simulink model "Mission_Server_QDrone_YOLO_Landing_Diagnostics"  (R2021b)
settings: Solver=ode2  StartTime=0.0  StopTime=inf  FixedStep=0.001  RelTol=1e-3  EnableMultiTasking=on
undefined symbols (not defined in the file): Host, qc_get_step_size
libraries: quarc_library x21, simulink x4
settings Model: SimulationMode=external  ExtModeTrigDuration=10000  Creator=Admin  LastModifiedBy=user
settings SolverCC: AlgebraicLoopSolver=TrustRegion  PositivePriorityOrder=on
settings DataIOCC: ReturnWorkspaceOutputs=off
settings DebuggingCC: SFUnexpectedBacktrackingDiag=warning  SFNoUnconditionalDefaultTransitionDiag=warning  SFExecutionAtInitializationDiag=none  SFMachineParentedDataDiag=warning  ArithmeticOperatorsInVariantConditions=warning
settings SFSimCC: SimUseLocalCustomCode=off  CustomCodeUndefinedFunction=UseInterfaceOnly
settings RTWCC: Description=QUARC Win64 Target Using Toolchain  SystemTargetFile=quarc_win64.tlc  TemplateMakefile=quarc_default_tmf  RTWUseLocalCustomCode=off  Toolchain=QUARC win64 | nmake (64-bit Windows)  BuildConfiguration=Faster Runs
settings CodeAppCC: StateflowObjectComments=on
settings STFCustomTargetCC: ConcurrentExecutionCompliant=on  UseToolchainInfoCompliant=on  SystemTargetFile=quarc_win64.tlc
settings GRTTargetCC: TargetLangStandard=C89/C90 (ANSI)  ParMdlRefBuildCompliant=off  CompOptLevelCompliant=off  CombineOutputUpdateFcns=off  MatFileLogging=off  CPPClassGenCompliant=off  GRTInterface=on  ExtMode=on  ExtModeMexFile=quarc_comm  ExtModeMexArgs='-w -d %d -uri %u -URI_Follower tcpip://localhost:18001'
settings ConfigComp: CovMetricSettings=dw  CovSaveCumulativeToWorkspaceVar=on  CovSaveSingleToWorkspaceVar=on  CovExternalEMLEnable=off

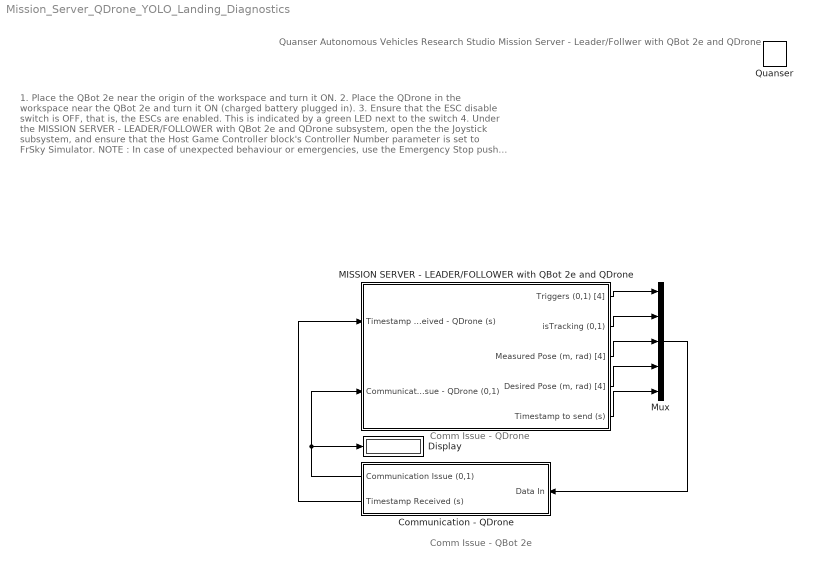
== system Mission_Server_QDrone_YOLO_Landing_Diagnostics ==
  note: 1. Place the QBot 2e near the origin of the workspace and turn it ON.
      | 2. Place the QDrone in the workspace near the QBot 2e and turn it ON (charged battery plugged in).
      | 3. Ensure that the ESC disable switch is OFF, that is, the ESCs are enabled. This is indicated by a green LED next to the switch
      | 4. Under the MISSION SERVER - LEADER/FOLLOWER with QBot 2e and QDrone subsystem, open the the Joystick subsystem, and ensure that the Host Game Controller block's Controller Number parameter is set to FrSky Simulator.
      | NOTE : In case of unexpected behaviour or emergencies, use the Emergency Stop push button on the Spektrum Joystick to cut all power to the motors (this will result in the drone falling).
      | 5. Open the Data Server (Localization) subsystem and follow the steps there to set up the correct calibration and rigid body definition files for the selected QBot 2e and QDrone.
      | 6. Under the QUARC menu, click on Build .
      | 7. Under the QUARC menu, click on Start . Wait for the model to start running (takes ~1 to 5 seconds for the Motive API to initialize and send localization data).
      | 8. In the MISSION SERVER - LEADER/FOLLOWER with QBot 2e and QDrone subsystem, ensure that the isTracking? display shows 1 and that the Joystick Issue display shows 0 (joystick must be powered ON with USB dongle attached to the PC).
      | 9. Start running the Joystick_Stabilizer_QBot2e_Leader.mdl model.
      | 10. Start running the Commander_Stabilizer_QDrone_Follower.mdl model.
      | 11. Arm the drone by moving the Arm/Disarm toggle to the 2 position.
      | 12. Takeoff the drone by moving the Takeoff/Land toggle to the 2 position. The QDrone should takeoff and hover.
      | 13. Drive the QBot 2e around using the joystick handset. Use the RIGHT stick (Roll/Pitch) to drive the QBot 2e forward/backward and turning/yawing.
      | 14. When finished, move the Takeoff/Land toggle to the 0 position to land the drone. The QDrone should land.
      | 15. Move the Arm/Disarm toggle to the 0 position. (the Commander_Stabilizer_QDrone_Follower.mdl model disarms the drone and stops automatically upon landing).
      | 16. Stop the QBot 2e model. Then stop this model.
  note: Quanser Autonomous Vehicles Research Studio
      | Mission Server - Leader/Follwer with QBot 2e and QDrone
  note: Comm Issue - QDrone
  note: Comm Issue - QBot 2e
  Communication - QDrone : Subsystem
  Display : Display
  MISSION SERVER - LEADER/FOLLOWER with QBot 2e and QDrone : Subsystem
  Mux : Mux  Inputs=5
  Quanser : quarc_library/Logos/Quanser
  wires:
  Communication - QDrone/2(Timestamp Received (s)) -> MISSION SERVER - LEADER/FOLLOWER with QBot 2e and QDrone/1(Timestamp Received - QDrone (s))
  MISSION SERVER - LEADER/FOLLOWER with QBot 2e and QDrone/5(Timestamp to send (s)) -> Mux/5
  Mux/1 -> Communication - QDrone/1(Data In)
  Communication - QDrone/1(Communication Issue (0,1)) -> Display/1, MISSION SERVER - LEADER/FOLLOWER with QBot 2e and QDrone/2(Communication Issue - QDrone (0,1))
  MISSION SERVER - LEADER/FOLLOWER with QBot 2e and QDrone/3("Measured Pose (m, rad) [4]") -> Mux/3
  MISSION SERVER - LEADER/FOLLOWER with QBot 2e and QDrone/4("Desired Pose (m, rad) [4]") -> Mux/4
  MISSION SERVER - LEADER/FOLLOWER with QBot 2e and QDrone/1(Triggers (0,1) [4]) -> Mux/1
  MISSION SERVER - LEADER/FOLLOWER with QBot 2e and QDrone/2(isTracking (0,1)) -> Mux/2

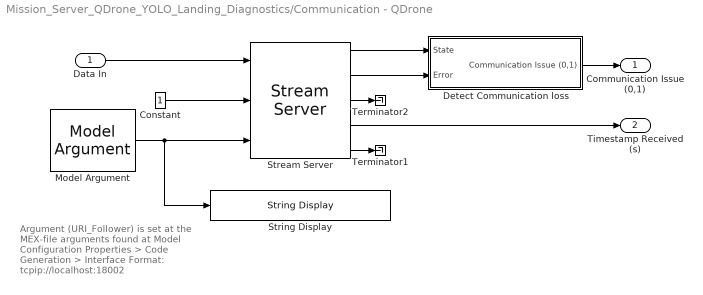
== system Mission_Server_QDrone_YOLO_Landing_Diagnostics/Communication - QDrone ==
  note: Argument (URI_Follower) is set at the MEX-file arguments found at Model Configuration Properties > Code Generation > Interface
      |
      | Format:
      | tcpip://localhost:18002
  Data In : Inport
  Constant : Constant
  Detect Communication loss : Subsystem
  Model Argument : quarc_library/Sources/Signals/Model Argument  argument_name=URI_Follower  has_value=on  data_type_mode=Specify via dialog  data_type=char  max_length=80  default_value=0  variable_size=off
      settings: AttributesFormatString=(-%<argument_name>)  SourceProductName=QUARC Targets
  Stream Server : quarc_library/Communications/Basic/Stream Server  uri_source=External input port  uri=tcpip://localhost:18877  send_buffer_size=1460  receive_buffer_size=1460  byte_order=little endian (Intel - LSB first)  optimization=Minimum latency  send_options=Send most recent data  receive_options=Receive most recent data  default_value=zeros(1,1)  sample_time=qc_get_step_size  active=off  implementation=Use blocking I/O in a separate thread  send_fifo_size=1000  receive_fifo_size=1000  send_priority=0  receive_priority=0  send_dimensions=off  receive_dimensions=off  max_dimensions=-1  data_type=Inherited via back propagation  type_expr=BusObject
  "String Display " : quarc_library/Strings/String Display  alignment=center  display_mode=Single line  sample_time=-1  use_new=off
      settings: SourceProductName=QUARC Targets
  Terminator1 : Terminator
  Terminator2 : Terminator
  Communication Issue (0,1) : Outport  VectorParamsAs1DForOutWhenUnconnected=off
  Timestamp Received (s) : Outport  Port=2  VectorParamsAs1DForOutWhenUnconnected=off
  wires:
  Constant/1 -> Stream Server/2
  Data In/1 -> Stream Server/1
  Stream Server/3 -> Terminator2/1
  Stream Server/5 -> Terminator1/1
  Model Argument/1 -> "String Display "/1, Stream Server/3
  Stream Server/4 -> Timestamp Received (s)/1
  Stream Server/1 -> Detect Communication loss/1(State)
  Stream Server/2 -> Detect Communication loss/2(Error)
  Detect Communication loss/1(Communication Issue (0,1)) -> Communication Issue (0,1)/1

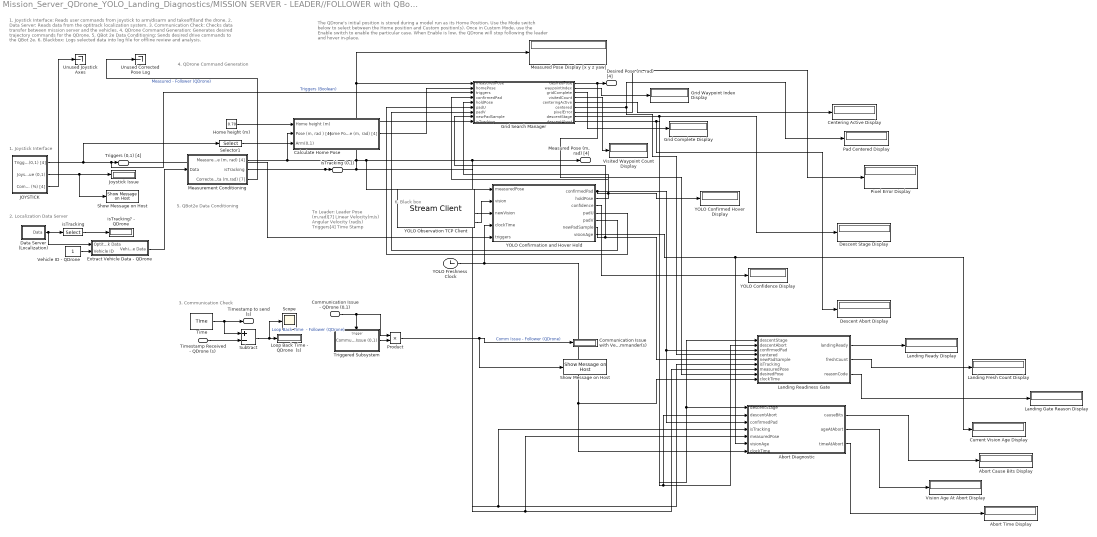
== system Mission_Server_QDrone_YOLO_Landing_Diagnostics/MISSION SERVER - LEADER//FOLLOWER with QBot 2e and QDrone ==
  note: To Leader:
      | Leader Pose (m,rad)[7]
      | Linear Velocity(m/s)
      | Angular Velocity (rad/s)
      | Triggers[4]
      | Time Stamp
  note: 5. QBot2e Data Conditioning
  note: The QDrone's initial position is stored during a model run as its Home Position.
      | Use the Mode switch below to select between the Home position and Custom position(s).
      | Once in Custom Mode, use the Enable switch to enable the particular case.
      | When Enable is low, the QDrone will stop following the leader and hover in-place.
  note: 3. Communication Check
  note: 6. Black box
  note: 2. Localization Data Server
  note: 1. Joystick Interface
  note: 4. QDrone Command Generation
  note: 1. Joystick Interface: Reads user commands from joystick to arm/disarm and takeoff/land the drone.
      | 2. Data Server: Reads data from the optitrack localization system.
      | 3. Communication Check: Checks data transfer between mission server and the vehicles.
      | 4. QDrone Command Generation: Generates desired trajectory commands for the QDrone.
      | 5. QBot 2e Data Conditioning: Sends desired drive commands to the QBot 2e.
      | 6. Blackbox: Logs selected data into log file for offline review and analysis.
  Timestamp Received - QDrone (s) : Inport
  Communication Issue - QDrone (0,1) : Inport  Port=2
  Abort Cause Bits Display : Display
  Abort Diagnostic : MATLAB Function  TreatAsAtomicUnit=on
  Abort Time Display : Display
  Calculate Home Pose : Subsystem
  Centering Active Display : Display
  Communication Issue with Vehicle Commander(s) : Display
  Current Vision Age Display : Display
  "Data Server (Localization) " : Subsystem
  Descent Abort Display : Display
  Descent Stage Display : Display
  Extract Vehicle Data - QDrone : Subsystem
  Grid Complete Display : Display
  Grid Search Manager : MATLAB Function  TreatAsAtomicUnit=on
  Grid Waypoint Index Display : Display
  Home height (m) : Constant  Value=0.70
  JOYSTICK : Subsystem
  Joystick Issue : Display
  Landing Fresh Count Display : Display
  Landing Gate Reason Display : Display
  Landing Readiness Gate : MATLAB Function  TreatAsAtomicUnit=on
  Landing Ready Display : Display
  Loop Back Time - QDrone  (s) : Display
  Measured Pose Display [x y z yaw] : Display
  Measurement Conditioning : Subsystem
  Pad Centered Display : Display
  Pixel Error Display : Display
  Product : Product
  Scope : Scope
  Selector1 : Selector  InputPortWidth=4  IndexOptions=Index vector (dialog)  Indices=[1]  OutputSizes=1
  Show Message on Host : quarc_library/Sinks/Error Handling/Show Message on Host  message_type=Fixed error message  message_icon=Warning  message=Mission Server: Communication Issue with remote vehicle(s)
      settings: AttributesFormatString="\"%<message>\""  SourceProductName=QUARC Targets
  "Show Message on Host " : quarc_library/Sinks/Error Handling/Show Message on Host  message_type=Fixed error message  message_icon=Warning  message=Mission Server: Joystick Disconnected
      settings: AttributesFormatString="\"%<message>\""  SourceProductName=QUARC Targets
  Subtract : Sum  Inputs=+-
  Time : quarc_library/Sources/Time/Time  time_source=Wall clock  sample_time=qc_get_step_size
  Triggered Subsystem : Subsystem  TreatAsAtomicUnit=on
  Unused Corrected Pose Log : Terminator
  Unused Joystick Axes : Terminator
  Vehicle ID - QDrone : Constant
  Vision Age At Abort Display : Display
  Visited Waypoint Count Display : Display
  YOLO Confidence Display : Display
  YOLO Confirmation and Hover Hold : MATLAB Function  TreatAsAtomicUnit=on
  YOLO Confirmed Hover Display : Display
  YOLO Freshness Clock : Clock
  YOLO Observation TCP Client : quarc_library/Communications/Basic/Stream Client  uri_source=Specify via dialog (do not evaluate)  uri=tcpip://localhost:18901  send_buffer_size=1460  receive_buffer_size=1460  byte_order=little endian (Intel - LSB first)  optimization=Minimum latency  send_options=Do not send data  receive_options=Receive most recent data  default_value=[0 0 0 0 -1 0]  sample_time=qc_get_step_size  active=off  implementation=Use blocking I/O in a separate thread  send_fifo_size=1000  receive_fifo_size=1000  send_priority=0  receive_priority=0  send_dimensions=off  receive_dimensions=off  max_dimensions=-1  data_type=Inherited via back propagation  type_expr=BusObject
      settings: AttributesFormatString="\"tcpip://localhost:18901\""
  isTracking : Selector  InputPortWidth=7  IndexOptions=Index vector (dialog)  Indices=[7]  OutputSizes=1
  isTracking? - QDrone : Display
  Triggers (0,1) [4] : Outport  VectorParamsAs1DForOutWhenUnconnected=off
  isTracking (0,1) : Outport  Port=2  VectorParamsAs1DForOutWhenUnconnected=off
  "Measured Pose (m, rad) [4]" : Outport  Port=3  VectorParamsAs1DForOutWhenUnconnected=off
  "Desired Pose (m, rad) [4]" : Outport  Port=4  VectorParamsAs1DForOutWhenUnconnected=off
  Timestamp to send (s) : Outport  Port=5  VectorParamsAs1DForOutWhenUnconnected=off
  wires:
  Communication Issue - QDrone (0,1)/1 -> Product/1, Triggered Subsystem/Trigger
  isTracking/1 -> isTracking? - QDrone/1
  JOYSTICK/2(Joystick Issue (0,1)) -> Joystick Issue/1, "Show Message on Host "/1
  Time/1 -> Timestamp to send (s)/1, Subtract/1
  Timestamp Received - QDrone (s)/1 -> Subtract/2
  Subtract/1 -> Loop Back Time - QDrone  (s)/1, Scope/1  "Loop Back Time  - Follower (QDrone)"
  Measurement Conditioning/2(isTracking) -> Landing Readiness Gate/6(isTracking), Abort Diagnostic/4(isTracking), Grid Search Manager/9(isTracking), isTracking (0,1)/1
  Measurement Conditioning/1("Measured Pose (m, rad) [4]") -> Landing Readiness Gate/7(measuredPose), Abort Diagnostic/5(measuredPose), "Measured Pose (m, rad) [4]"/1, YOLO Confirmation and Hover Hold/1(measuredPose), Measured Pose Display [x y z yaw]/1, Grid Search Manager/1(measuredPose), Calculate Home Pose/2("Pose (m, rad ) [4]")
  "Data Server (Localization) "/1(Data) -> isTracking/1, Extract Vehicle Data - QDrone/1(Optitrack Data)
  Vehicle ID - QDrone/1 -> Extract Vehicle Data - QDrone/2(Vehicle ID)
  Calculate Home Pose/1("Home Pose (m, rad) [4]") -> Grid Search Manager/2(homePose)
  Home height (m)/1 -> Calculate Home Pose/1(Home height (m))
  Triggered Subsystem/1(Communication Issue (0,1)) -> Product/2
  Product/1 -> Communication Issue with Vehicle Commander(s)/1, Show Message on Host/1  "Comm Issue - Follower (QDrone)"
  Extract Vehicle Data - QDrone/1(Vehicle Data) -> Measurement Conditioning/1(Data)
  JOYSTICK/1(Triggers (0,1) [4]) -> YOLO Confirmation and Hover Hold/5(triggers), Grid Search Manager/3(triggers), Triggers (0,1) [4]/1, Selector1/1  "Triggers (Boolean)"
  JOYSTICK/3(Commands (%) [4]) -> Unused Joystick Axes/1
  Selector1/1 -> Calculate Home Pose/3(Arm(0,1))
  Measurement Conditioning/3(Corrected Pose Data (m,rad) [7]) -> Unused Corrected Pose Log/1  "Measured - Follower (QDrone)"
  Grid Search Manager/1(desiredPose) -> "Desired Pose (m, rad) [4]"/1, Landing Readiness Gate/8(desiredPose)
  Grid Search Manager/2(waypointIndex) -> Grid Waypoint Index Display/1
  Grid Search Manager/3(gridComplete) -> Grid Complete Display/1
  Grid Search Manager/4(visitedCount) -> Visited Waypoint Count Display/1
  YOLO Observation TCP Client/3 -> YOLO Confirmation and Hover Hold/2(vision)
  YOLO Observation TCP Client/4 -> YOLO Confirmation and Hover Hold/3(newVision)
  YOLO Freshness Clock/1 -> Abort Diagnostic/7(clockTime), Landing Readiness Gate/9(clockTime), YOLO Confirmation and Hover Hold/4(clockTime)
  YOLO Confirmation and Hover Hold/1(confirmedPad) -> Landing Readiness Gate/3(confirmedPad), Abort Diagnostic/3(confirmedPad), Grid Search Manager/4(confirmedPad), YOLO Confirmed Hover Display/1
  YOLO Confirmation and Hover Hold/2(holdPose) -> Grid Search Manager/5(holdPose)
  YOLO Confirmation and Hover Hold/3(confidence) -> YOLO Confidence Display/1
  YOLO Confirmation and Hover Hold/4(padU) -> Grid Search Manager/6(padU)
  YOLO Confirmation and Hover Hold/5(padV) -> Grid Search Manager/7(padV)
  YOLO Confirmation and Hover Hold/6(newPadSample) -> Grid Search Manager/8(newPadSample), Landing Readiness Gate/5(newPadSample)
  Grid Search Manager/5(centeringActive) -> Centering Active Display/1
  Grid Search Manager/6(centered) -> Pad Centered Display/1, Landing Readiness Gate/4(centered)
  Grid Search Manager/7(pixelError) -> Pixel Error Display/1
  Grid Search Manager/8(descentStage) -> Landing Readiness Gate/1(descentStage), Abort Diagnostic/1(descentStage), Descent Stage Display/1
  Grid Search Manager/9(descentAbort) -> Abort Diagnostic/2(descentAbort), Landing Readiness Gate/2(descentAbort), Descent Abort Display/1
  Landing Readiness Gate/1(landingReady) -> Landing Ready Display/1
  Landing Readiness Gate/2(freshCount) -> Landing Fresh Count Display/1
  Landing Readiness Gate/3(reasonCode) -> Landing Gate Reason Display/1
  YOLO Confirmation and Hover Hold/7(visionAge) -> Abort Diagnostic/6(visionAge), Current Vision Age Display/1
  Abort Diagnostic/1(causeBits) -> Abort Cause Bits Display/1
  Abort Diagnostic/2(ageAtAbort) -> Vision Age At Abort Display/1
  Abort Diagnostic/3(timeAtAbort) -> Abort Time Display/1

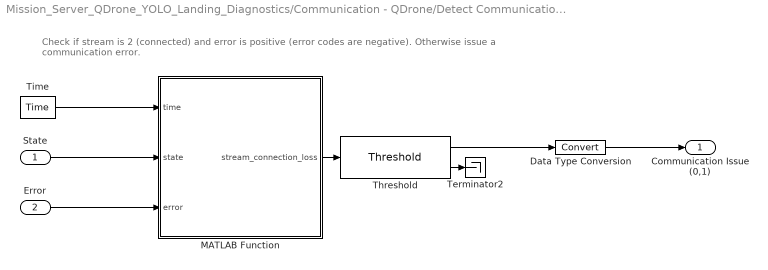
== system Mission_Server_QDrone_YOLO_Landing_Diagnostics/Communication - QDrone/Detect Communication loss ==
  note: Check if stream is 2 (connected) and error is positive (error codes are negative). Otherwise issue a communication error.
  State : Inport
  Error : Inport  Port=2
  Data Type Conversion : DataTypeConversion
  MATLAB Function : MATLAB Function  TreatAsAtomicUnit=on
  Terminator2 : Terminator
  Threshold : quarc_library/Discontinuities/Threshold  operator=>=  param_src=Specify via dialog  threshold=0.5  duration=0.1
      settings: SourceProductName=QUARC Targets
  Time : quarc_library/Sources/Time/Time  time_source=Wall clock  sample_time=qc_get_step_size
  Communication Issue (0,1) : Outport  VectorParamsAs1DForOutWhenUnconnected=off
  wires:
  Error/1 -> MATLAB Function/3(error)
  MATLAB Function/1(stream_connection_loss) -> Threshold/1
  State/1 -> MATLAB Function/2(state)
  Time/1 -> MATLAB Function/1(time)
  Threshold/2 -> Terminator2/1
  Data Type Conversion/1 -> Communication Issue (0,1)/1
  Threshold/1 -> Data Type Conversion/1

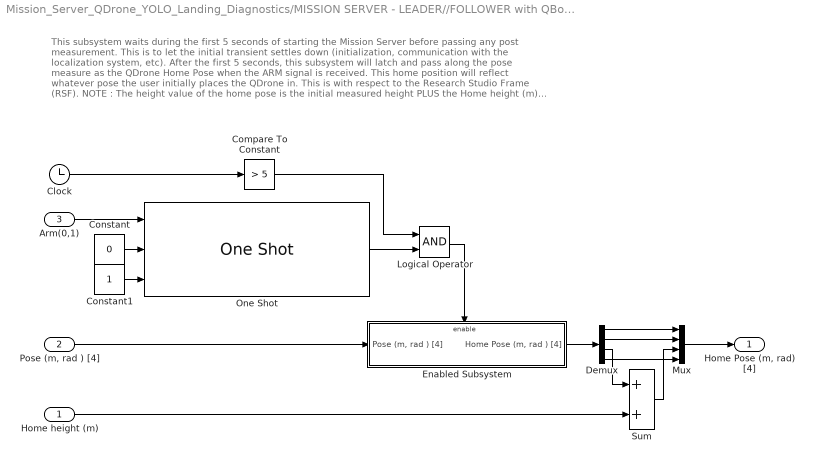
== system Mission_Server_QDrone_YOLO_Landing_Diagnostics/MISSION SERVER - LEADER//FOLLOWER with QBot 2e and QDrone/Calculate Home Pose ==
  note: This subsystem waits during the first 5 seconds of starting the Mission Server before passing any post measurement.
      | This is to let the initial transient settles down (initialization, communication with the localization system, etc).
      | After the first 5 seconds, this subsystem will latch and pass along the pose measure as the QDrone Home Pose when
      | the ARM signal is received.
      | This home position will reflect whatever pose the user initially places the QDrone in.
      | This is with respect to the Research Studio Frame (RSF).
      |
      | NOTE : The height value of the home pose is the initial measured height PLUS the Home height (m) input value.
  Home height (m) : Inport
  "Pose (m, rad ) [4]" : Inport  Port=2
  Arm(0,1) : Inport  Port=3
  Clock : Clock
  Compare To Constant : simulink/Logic and Bit Operations/Compare To Constant  relop=>  const=5  OutDataTypeStr=boolean
  Constant : Constant  Value=0
  Constant1 : Constant
  Demux : Demux
  Enabled Subsystem : Subsystem  TreatAsAtomicUnit=on
  Logical Operator : Logic  AllPortsSameDT=off  OutDataTypeStr=boolean
  Mux : Mux
  One Shot : quarc_library/Discontinuities/One Shot  trigger_type=Rising edge  redun_pulse=Ignore extraneous pulse  width_source=Specify via dialog  pulse_width=1/qc_get_step_size
      settings: SourceProductName=QUARC Targets
  Sum : Sum
  "Home Pose (m, rad) [4]" : Outport  VectorParamsAs1DForOutWhenUnconnected=off
  wires:
  Constant/1 -> One Shot/2
  Constant1/1 -> One Shot/3
  Arm(0,1)/1 -> One Shot/1
  One Shot/1 -> Logical Operator/2
  "Pose (m, rad ) [4]"/1 -> Enabled Subsystem/1("Pose (m, rad ) [4] ")
  Clock/1 -> Compare To Constant/1
  Compare To Constant/1 -> Logical Operator/1
  Logical Operator/1 -> Enabled Subsystem/Enable
  Enabled Subsystem/1("Home Pose (m, rad ) [4]") -> Demux/1
  Demux/1 -> Mux/1
  Demux/2 -> Mux/2
  Demux/4 -> Mux/4
  Demux/3 -> Sum/1
  Sum/1 -> Mux/3
  Home height (m)/1 -> Sum/2
  Mux/1 -> "Home Pose (m, rad) [4]"/1

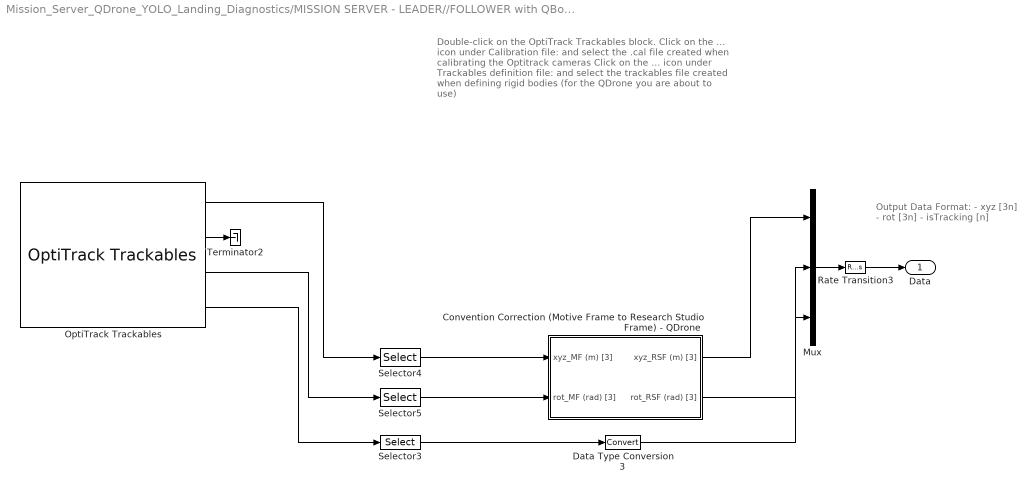
== system Mission_Server_QDrone_YOLO_Landing_Diagnostics/MISSION SERVER - LEADER//FOLLOWER with QBot 2e and QDrone/Data Server (Localization)  ==
  note: Output Data Format:
      | - xyz [3n]
      | - rot [3n]
      | - isTracking [n]
  note: Double-click on the OptiTrack Trackables block.
      |
      | Click on the ... icon under Calibration file: and select the .cal file
      | created when calibrating the Optitrack cameras
      |
      | Click on the ... icon under Trackables definition file: and select
      | the trackables file created when defining rigid bodies (for the
      | QDrone you are about to use)
  Convention Correction (Motive Frame to Research Studio Frame) - QDrone : Subsystem
  Data Type Conversion3 : DataTypeConversion
  Mux : Mux  Inputs=3
  OptiTrack Trackables : quarc_library/Devices/Third-Party/NaturalPoint/OptiTrack/OptiTrack Trackables  calibration_file=C:\Users\user\Documents\OptiTrack\Session 2026-09-15\Calibration Exceptional (MeanErr 0.544 mm) 2026-09-15 10.cal  rigid_body_file=C:\Users\user\Documents\OptiTrack\Session 2026-09-15\RigidBody 01.tra  rigid_body_ids=1  sample_time=qc_get_step_size*10  active=off
      settings: SourceProductName=QUARC Targets
  Rate Transition3 : RateTransition
  Selector3 : Selector  InputPortWidth=1  IndexOptions=Index vector (dialog)  Indices=[1]  OutputSizes=1
  Selector4 : Selector  InputPortWidth=3  IndexOptions=Index vector (dialog)  Indices=[1:3]  OutputSizes=1
  Selector5 : Selector  InputPortWidth=3  IndexOptions=Index vector (dialog)  Indices=[1:3]  OutputSizes=1
  Terminator2 : Terminator
  Data : Outport  VectorParamsAs1DForOutWhenUnconnected=off
  wires:
  OptiTrack Trackables/2 -> Terminator2/1
  OptiTrack Trackables/4 -> Selector3/1
  OptiTrack Trackables/3 -> Selector5/1
  Selector3/1 -> Data Type Conversion3/1
  OptiTrack Trackables/1 -> Selector4/1
  Selector4/1 -> Convention Correction (Motive Frame to Research Studio Frame) - QDrone/1(xyz_MF (m) [3])
  Selector5/1 -> Convention Correction (Motive Frame to Research Studio Frame) - QDrone/2(rot_MF (rad) [3])
  Mux/1 -> Rate Transition3/1
  Rate Transition3/1 -> Data/1
  Convention Correction (Motive Frame to Research Studio Frame) - QDrone/1(xyz_RSF (m) [3]) -> Mux/1
  Convention Correction (Motive Frame to Research Studio Frame) - QDrone/2(rot_RSF (rad) [3]) -> Mux/2
  Data Type Conversion3/1 -> Mux/3

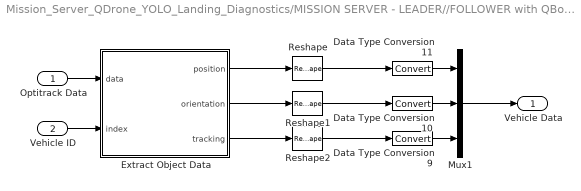
== system Mission_Server_QDrone_YOLO_Landing_Diagnostics/MISSION SERVER - LEADER//FOLLOWER with QBot 2e and QDrone/Extract Vehicle Data - QDrone ==
  Optitrack Data : Inport
  Vehicle ID : Inport  Port=2
  Data Type Conversion10 : DataTypeConversion
  Data Type Conversion11 : DataTypeConversion
  Data Type Conversion9 : DataTypeConversion
  Extract Object Data : MATLAB Function  TreatAsAtomicUnit=on
  Mux1 : Mux  Inputs=3
  Reshape : Reshape
  Reshape1 : Reshape
  Reshape2 : Reshape
  Vehicle Data : Outport  VectorParamsAs1DForOutWhenUnconnected=off
  wires:
  Reshape2/1 -> Data Type Conversion9/1
  Reshape1/1 -> Data Type Conversion10/1
  Reshape/1 -> Data Type Conversion11/1
  Data Type Conversion9/1 -> Mux1/3
  Data Type Conversion10/1 -> Mux1/2
  Data Type Conversion11/1 -> Mux1/1
  Extract Object Data/2(orientation) -> Reshape1/1
  Extract Object Data/3(tracking) -> Reshape2/1
  Extract Object Data/1(position) -> Reshape/1
  Mux1/1 -> Vehicle Data/1
  Optitrack Data/1 -> Extract Object Data/1(data)
  Vehicle ID/1 -> Extract Object Data/2(index)

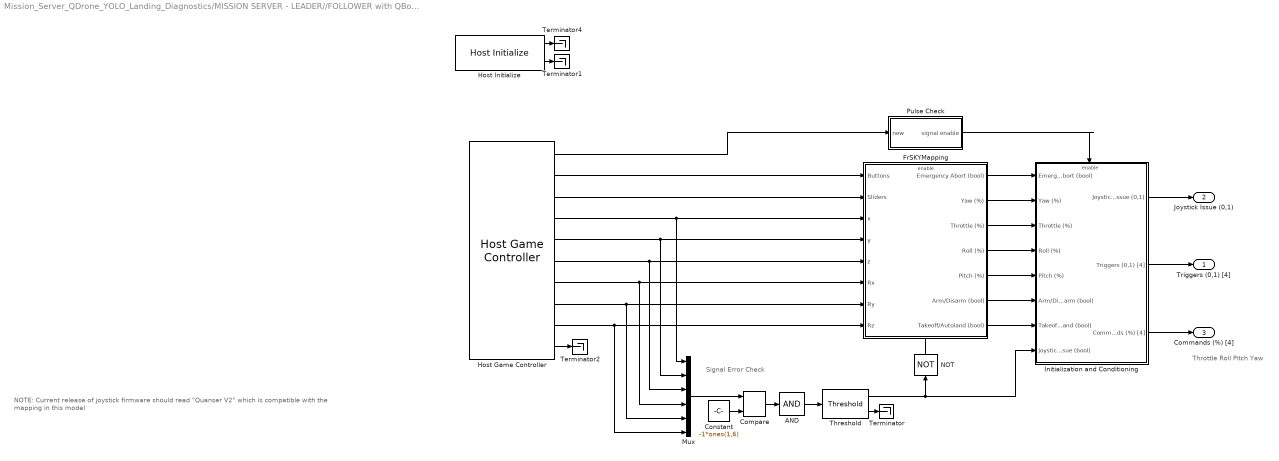
== system Mission_Server_QDrone_YOLO_Landing_Diagnostics/MISSION SERVER - LEADER//FOLLOWER with QBot 2e and QDrone/JOYSTICK ==
  note: Throttle
      | Roll
      | Pitch
      | Yaw
  note: Signal Error Check
  note: NOTE: Current release of joystick firmware should read "Quanser V2" which is compatible with the mapping in this model
  AND : Logic  Inputs=1  AllPortsSameDT=off  OutDataTypeStr=boolean
  Compare : quarc_library/Logic Operations/Compare  operator===  output_data_type=boolean
      settings: SourceProductName=QUARC Targets
  Constant : Constant  Value=-1*ones(1,6)
  FrSKYMapping : Subsystem
  Host Game Controller : quarc_library/Devices/Peripherals/Host/Host Game Controller  object_name=Host-1  controller=1  buffer_size=20  deadzone=[]  saturation=[]  sample_time=qc_get_step_size  auto_center=off  enabled=on  debug_mode=off
      settings: SourceProductName=QUARC Targets
  Host Initialize : quarc_library/Devices/Peripherals/Host/Host Initialize  object_name=Host-1  uri_source=Use external mode communications  uri=tcpip://localhost:18001  send_buffer_size=1000  receive_buffer_size=1000  thread_priority=0  run_client=on  use_window=off  window_position=[]  sample_time=qc_get_step_size  active=on
      settings: SourceProductName=QUARC Targets
  Initialization and Conditioning : Subsystem  TreatAsAtomicUnit=on
  Mux : Mux  Inputs=6
  NOT : Logic  Operator=NOT  IconShape=distinctive  AllPortsSameDT=off  OutDataTypeStr=boolean
  Pulse Check : Subsystem  TreatAsAtomicUnit=on
  Terminator{,1..2,4} (4 alike) : Terminator
  Threshold : quarc_library/Discontinuities/Threshold  operator=>=  param_src=Specify via dialog  threshold=0.5  duration=0.2
      settings: SourceProductName=QUARC Targets
  Triggers (0,1) [4] : Outport  VectorParamsAs1DForOutWhenUnconnected=off
  Joystick Issue (0,1) : Outport  Port=2  VectorParamsAs1DForOutWhenUnconnected=off
  Commands (%) [4] : Outport  Port=3  VectorParamsAs1DForOutWhenUnconnected=off
  wires:
  Initialization and Conditioning/1(Joystick Issue (0,1)) -> Joystick Issue (0,1)/1
  Host Game Controller/10 -> Terminator2/1
  Host Initialize/1 -> Terminator4/1
  Host Initialize/2 -> Terminator1/1
  Initialization and Conditioning/2(Triggers (0,1) [4]) -> Triggers (0,1) [4]/1
  Initialization and Conditioning/3(Commands (%) [4]) -> Commands (%) [4]/1
  AND/1 -> Threshold/1
  NOT/1 -> FrSKYMapping/Enable
  Threshold/1 -> Initialization and Conditioning/8(Joystick Issue (bool)), NOT/1
  Host Game Controller/3 -> FrSKYMapping/2(Sliders)
  Host Game Controller/2 -> FrSKYMapping/1(Buttons)
  Threshold/2 -> Terminator/1
  Compare/1 -> AND/1
  Constant/1 -> Compare/2
  Mux/1 -> Compare/1
  Host Game Controller/9 -> FrSKYMapping/8(Rz), Mux/6
  Host Game Controller/8 -> FrSKYMapping/7(Ry), Mux/5
  Host Game Controller/7 -> FrSKYMapping/6(Rx), Mux/4
  Host Game Controller/6 -> FrSKYMapping/5(z), Mux/3
  Host Game Controller/5 -> FrSKYMapping/4(y), Mux/2
  Host Game Controller/4 -> FrSKYMapping/3(x), Mux/1
  FrSKYMapping/7(Takeoff/Autoland (bool)) -> Initialization and Conditioning/7(Takeoff/AutoLand (bool))
  Pulse Check/1(signal enable) -> Initialization and Conditioning/Enable
  Host Game Controller/1 -> Pulse Check/1(new)
  FrSKYMapping/4(Roll (%)) -> Initialization and Conditioning/4(Roll (%))
  FrSKYMapping/6("Arm/Disarm (bool) ") -> Initialization and Conditioning/6(Arm/Disarm (bool))
  FrSKYMapping/5(Pitch (%)) -> Initialization and Conditioning/5(Pitch (%))
  FrSKYMapping/1(Emergency Abort (bool)) -> Initialization and Conditioning/1(Emergency Abort (bool))
  FrSKYMapping/3(Throttle (%)) -> Initialization and Conditioning/3(Throttle (%))
  FrSKYMapping/2(Yaw (%)) -> Initialization and Conditioning/2(Yaw (%))

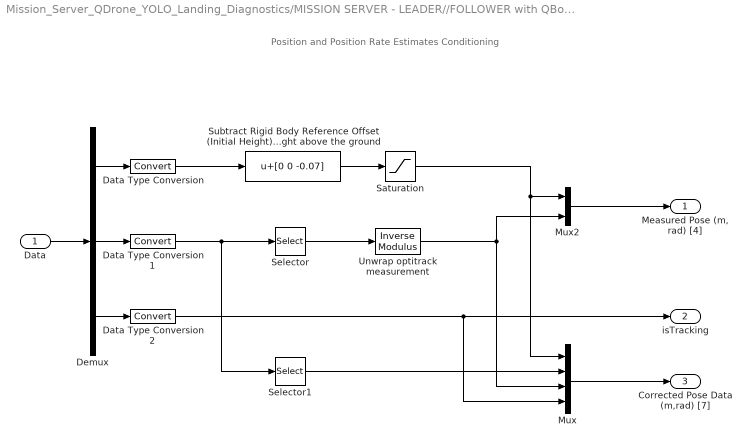
== system Mission_Server_QDrone_YOLO_Landing_Diagnostics/MISSION SERVER - LEADER//FOLLOWER with QBot 2e and QDrone/Measurement Conditioning ==
  note: Position and Position Rate Estimates Conditioning
  Data : Inport
  Data Type Conversion : DataTypeConversion
  Data Type Conversion1 : DataTypeConversion
  Data Type Conversion2 : DataTypeConversion
  Demux : Demux  Outputs=[3 3 1]
  Mux : Mux
  Mux2 : Mux  Inputs=[3 1]
  Saturation : Saturate  UpperLimit=[2 2 5]  LowerLimit=[-2 -2 0]
  Selector : Selector  InputPortWidth=3  IndexOptions=Index vector (dialog)  Indices=[3]  OutputSizes=1
  Selector1 : Selector  InputPortWidth=3  IndexOptions=Index vector (dialog)  Indices=[1 2]  OutputSizes=1
  Subtract Rigid Body Reference Offset (Initial Height) to get height above the ground : Bias  Bias=[0 0 -0.07]
  Unwrap optitrack measurement : quarc_library/Discontinuities/Inverse Modulus  modulus=2*pi  output_derivative=off  output_revolutions=off  max_x=Inf  min_x=-Inf
  "Measured Pose (m, rad) [4]" : Outport  VectorParamsAs1DForOutWhenUnconnected=off
  isTracking : Outport  Port=2  VectorParamsAs1DForOutWhenUnconnected=off
  Corrected Pose Data (m,rad) [7] : Outport  Port=3  VectorParamsAs1DForOutWhenUnconnected=off
  wires:
  Demux/2 -> Data Type Conversion1/1
  Demux/1 -> Data Type Conversion/1
  Demux/3 -> Data Type Conversion2/1
  Mux2/1 -> "Measured Pose (m, rad) [4]"/1
  Data/1 -> Demux/1
  Data Type Conversion2/1 -> Mux/4, isTracking/1
  Subtract Rigid Body Reference Offset (Initial Height) to get height above the ground/1 -> Saturation/1
  Saturation/1 -> Mux2/1, Mux/1
  Data Type Conversion1/1 -> Selector1/1, Selector/1
  Selector/1 -> Unwrap optitrack measurement/1
  Data Type Conversion/1 -> Subtract Rigid Body Reference Offset (Initial Height) to get height above the ground/1
  Unwrap optitrack measurement/1 -> Mux/3, Mux2/2
  Mux/1 -> Corrected Pose Data (m,rad) [7]/1
  Selector1/1 -> Mux/2

== system Mission_Server_QDrone_YOLO_Landing_Diagnostics/MISSION SERVER - LEADER//FOLLOWER with QBot 2e and QDrone/Triggered Subsystem ==
  note: This looks for the first falling edge of the communication issue before allowing a communication issue to be triggered,
      | because the mission server model starts first.
  Trigger : TriggerPort  TriggerType=falling  VariantControl=Variant
  Add : Sum
  Compare To Constant : simulink/Logic and Bit Operations/Compare To Constant  relop=>=  const=1  OutDataTypeStr=boolean
  Constant : Constant
  Memory : Memory  InheritSampleTime=on
  Communication Issue (0,1) : Outport  InitialOutput=0  VectorParamsAs1DForOutWhenUnconnected=off
  wires:
  Constant/1 -> Add/1
  Memory/1 -> Add/2
  Add/1 -> Compare To Constant/1, Memory/1
  Compare To Constant/1 -> Communication Issue (0,1)/1

== system Mission_Server_QDrone_YOLO_Landing_Diagnostics/MISSION SERVER - LEADER//FOLLOWER with QBot 2e and QDrone/Calculate Home Pose/Enabled Subsystem ==
  "Pose (m, rad ) [4] " : Inport
  Enable : EnablePort
  "Home Pose (m, rad ) [4]" : Outport  VectorParamsAs1DForOutWhenUnconnected=off
  wires:
  "Pose (m, rad ) [4] "/1 -> "Home Pose (m, rad ) [4]"/1

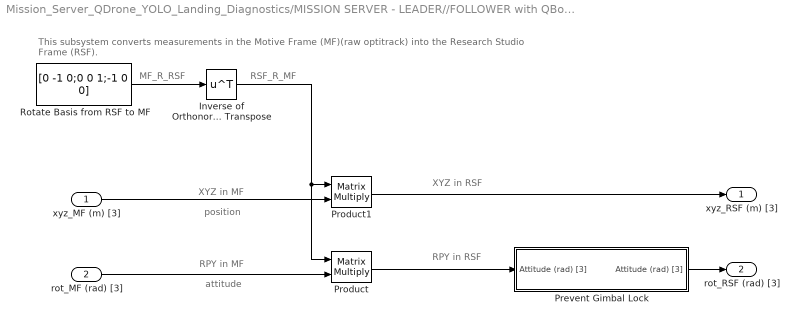
== system Mission_Server_QDrone_YOLO_Landing_Diagnostics/MISSION SERVER - LEADER//FOLLOWER with QBot 2e and QDrone/Data Server (Localization) /Convention Correction (Motive Frame to Research Studio Frame) - QDrone ==
  note: MF_R_RSF
  note: This subsystem converts measurements in the Motive Frame (MF)(raw optitrack) into the Research Studio Frame (RSF).
  note: RSF_R_MF
  note: XYZ in MF
  note: RPY in MF
  note: position
  note: attitude
  note: XYZ in RSF
  note: RPY in RSF
  xyz_MF (m) [3] : Inport
  rot_MF (rad) [3] : Inport  Port=2
  Inverse of Orthonormal Matrix is its Transpose : Math  Operator=transpose  SignedPower=on  SaturateOnIntegerOverflow=on
  Prevent Gimbal Lock : Subsystem
  Product : Product  Multiplication=Matrix(*)
  Product1 : Product  Multiplication=Matrix(*)
  Rotate Basis from RSF to MF : Constant  Value=[0 -1 0;0 0 1;-1 0 0]
  xyz_RSF (m) [3] : Outport  VectorParamsAs1DForOutWhenUnconnected=off
  rot_RSF (rad) [3] : Outport  Port=2  VectorParamsAs1DForOutWhenUnconnected=off
  wires:
  Rotate Basis from RSF to MF/1 -> Inverse of Orthonormal Matrix is its Transpose/1
  xyz_MF (m) [3]/1 -> Product1/2
  Inverse of Orthonormal Matrix is its Transpose/1 -> Product1/1, Product/1
  rot_MF (rad) [3]/1 -> Product/2
  Product1/1 -> xyz_RSF (m) [3]/1
  Product/1 -> Prevent Gimbal Lock/1(Attitude (rad) [3])
  Prevent Gimbal Lock/1("Attitude (rad) [3] ") -> rot_RSF (rad) [3]/1

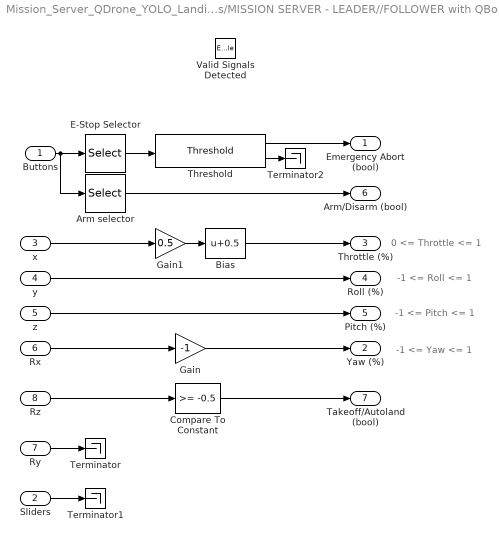
== system Mission_Server_QDrone_YOLO_Landing_Diagnostics/MISSION SERVER - LEADER//FOLLOWER with QBot 2e and QDrone/JOYSTICK/FrSKYMapping ==
  note: -1 <= Pitch <= 1
  note: -1 <= Roll <= 1
  note: 0 <= Throttle <= 1
  note: -1 <= Yaw <= 1
  Buttons : Inport
  Sliders : Inport  Port=2
  x : Inport  Port=3
  y : Inport  Port=4
  z : Inport  Port=5
  Rx : Inport  Port=6
  Ry : Inport  Port=7
  Rz : Inport  Port=8
  Valid Signals Detected : EnablePort
  Arm selector : Selector  InputPortWidth=32  IndexOptions=Index vector (dialog)  Indices=[2]  OutputSizes=1
  Bias : Bias  Bias=0.5
  Compare To Constant : simulink/Logic and Bit Operations/Compare To Constant  relop=>=  const=-0.5  OutDataTypeStr=boolean
  E-Stop Selector : Selector  InputPortWidth=32  IndexOptions=Index vector (dialog)  Indices=[1]  OutputSizes=1
  Gain : Gain  Gain=-1
  Gain1 : Gain  Gain=0.5
  Terminator : Terminator
  Terminator1 : Terminator
  Terminator2 : Terminator
  Threshold : quarc_library/Discontinuities/Threshold  operator=>=  param_src=Specify via dialog  threshold=0.5  duration=0.2
      settings: SourceProductName=QUARC Targets
  Emergency Abort (bool) : Outport  VectorParamsAs1DForOutWhenUnconnected=off
  Yaw (%) : Outport  Port=2  VectorParamsAs1DForOutWhenUnconnected=off
  Throttle (%) : Outport  Port=3  VectorParamsAs1DForOutWhenUnconnected=off
  Roll (%) : Outport  Port=4  VectorParamsAs1DForOutWhenUnconnected=off
  Pitch (%) : Outport  Port=5  VectorParamsAs1DForOutWhenUnconnected=off
  "Arm/Disarm (bool) " : Outport  Port=6  VectorParamsAs1DForOutWhenUnconnected=off
  Takeoff/Autoland (bool) : Outport  Port=7  VectorParamsAs1DForOutWhenUnconnected=off
  wires:
  Bias/1 -> Throttle (%)/1
  Gain1/1 -> Bias/1
  Gain/1 -> Yaw (%)/1
  Threshold/2 -> Terminator2/1
  Threshold/1 -> Emergency Abort (bool)/1
  Compare To Constant/1 -> Takeoff/Autoland (bool)/1
  Rz/1 -> Compare To Constant/1
  E-Stop Selector/1 -> Threshold/1
  Sliders/1 -> Terminator1/1
  Ry/1 -> Terminator/1
  Rx/1 -> Gain/1
  z/1 -> Pitch (%)/1
  y/1 -> Roll (%)/1
  x/1 -> Gain1/1
  Arm selector/1 -> "Arm/Disarm (bool) "/1
  Buttons/1 -> E-Stop Selector/1, Arm selector/1

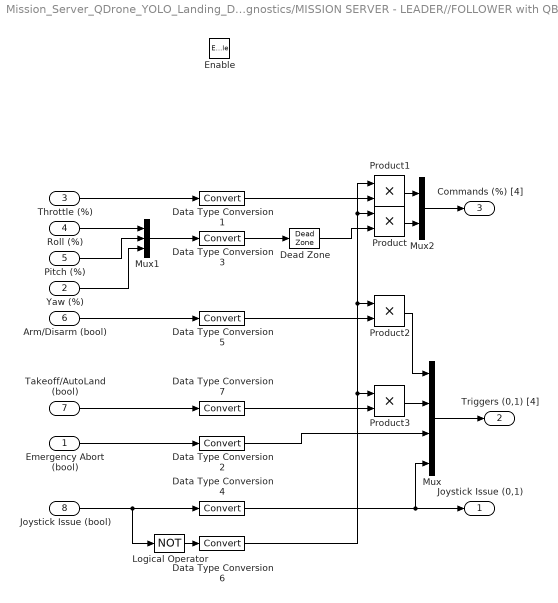
== system Mission_Server_QDrone_YOLO_Landing_Diagnostics/MISSION SERVER - LEADER//FOLLOWER with QBot 2e and QDrone/JOYSTICK/Initialization and Conditioning ==
  Emergency Abort (bool) : Inport
  Yaw (%) : Inport  Port=2
  Throttle (%) : Inport  Port=3
  Roll (%) : Inport  Port=4
  Pitch (%) : Inport  Port=5
  Arm/Disarm (bool) : Inport  Port=6
  Takeoff/AutoLand (bool) : Inport  Port=7
  Joystick Issue (bool) : Inport  Port=8
  Enable : EnablePort  StatesWhenEnabling=reset
  Data Type Conversion{1..7} (7 alike) : DataTypeConversion
  Dead Zone : DeadZone  LowerValue=-0.01  UpperValue=0.01  SaturateOnIntegerOverflow=on
  Logical Operator : Logic  Operator=NOT  AllPortsSameDT=off  OutDataTypeStr=boolean
  Mux : Mux
  Mux1 : Mux  Inputs=3
  Mux2 : Mux  Inputs=2
  Product{,1..3} (4 alike) : Product
  Joystick Issue (0,1) : Outport  InitialOutput=0  VectorParamsAs1DForOutWhenUnconnected=off
  Triggers (0,1) [4] : Outport  Port=2  InitialOutput=0  VectorParamsAs1DForOutWhenUnconnected=off
  Commands (%) [4] : Outport  Port=3  InitialOutput=0  VectorParamsAs1DForOutWhenUnconnected=off
  wires:
  Mux2/1 -> Commands (%) [4]/1
  Data Type Conversion7/1 -> Product3/2
  Product3/1 -> Mux/2
  Takeoff/AutoLand (bool)/1 -> Data Type Conversion7/1
  Data Type Conversion5/1 -> Product2/2
  Product2/1 -> Mux/1
  Data Type Conversion6/1 -> Product3/1, Product2/1, Product/1, Product1/1
  Dead Zone/1 -> Product/2
  Data Type Conversion1/1 -> Product1/2
  Product1/1 -> Mux2/1
  Product/1 -> Mux2/2
  Logical Operator/1 -> Data Type Conversion6/1
  Data Type Conversion2/1 -> Mux/3
  Mux/1 -> Triggers (0,1) [4]/1
  Arm/Disarm (bool)/1 -> Data Type Conversion5/1
  Data Type Conversion3/1 -> Dead Zone/1
  Emergency Abort (bool)/1 -> Data Type Conversion2/1
  Data Type Conversion4/1 -> Joystick Issue (0,1)/1, Mux/4
  Yaw (%)/1 -> Mux1/3
  Pitch (%)/1 -> Mux1/2
  Roll (%)/1 -> Mux1/1
  Throttle (%)/1 -> Data Type Conversion1/1
  Mux1/1 -> Data Type Conversion3/1
  Joystick Issue (bool)/1 -> Logical Operator/1, Data Type Conversion4/1

== system Mission_Server_QDrone_YOLO_Landing_Diagnostics/MISSION SERVER - LEADER//FOLLOWER with QBot 2e and QDrone/JOYSTICK/Pulse Check ==
  note: For this subsystem we will count the number of new pulses. The data can be considered enabled once the count of new signals has gone beyond 1. This will enable the Initializing and conditioning subsystem.
  new : Inport
  Compare : quarc_library/Logic Operations/Compare  operator=>=  output_data_type=boolean
      settings: SourceProductName=QUARC Targets
  Pulse Check : Constant
  "pulse count " : Subsystem  TreatAsAtomicUnit=on
  signal enable : Outport  InitialOutput=0  VectorParamsAs1DForOutWhenUnconnected=off
  wires:
  Compare/1 -> signal enable/1
  Pulse Check/1 -> Compare/2
  new/1 -> "pulse count "/Trigger
  "pulse count "/1(Number of Pulses) -> Compare/1

== system Mission_Server_QDrone_YOLO_Landing_Diagnostics/MISSION SERVER - LEADER//FOLLOWER with QBot 2e and QDrone/Data Server (Localization) /Convention Correction (Motive Frame to Research Studio Frame) - QDrone/Prevent Gimbal Lock ==
  note: Remapping the rotation order to prevent gimbal lock
      | in heading/yaw due to Euler singularity condition
  Attitude (rad) [3] : Inport
  Demux : Demux  Outputs=3
  Euler Angles from Rotation Matrix (Relative ZYX) : quarc_library/Math Operations/Matrices/Euler Angles from Rotation Matrix  menu_order=Relative Z-Y-X
      settings: SourceProductName=QUARC Targets
  Euler Angles to Rotation Matrix (Relative YZX) : quarc_library/Math Operations/Matrices/Euler Angles to Rotation Matrix  menu_order=Relative Y-Z-X
      settings: SourceProductName=QUARC Targets
  Mux : Mux  Inputs=3
  "Attitude (rad) [3] " : Outport  VectorParamsAs1DForOutWhenUnconnected=off
  wires:
  Euler Angles from Rotation Matrix (Relative ZYX)/2 -> Mux/2
  Euler Angles from Rotation Matrix (Relative ZYX)/1 -> Mux/3
  Euler Angles from Rotation Matrix (Relative ZYX)/3 -> Mux/1
  Euler Angles to Rotation Matrix (Relative YZX)/1 -> Euler Angles from Rotation Matrix (Relative ZYX)/1
  Attitude (rad) [3]/1 -> Demux/1
  Mux/1 -> "Attitude (rad) [3] "/1
  Demux/2 -> Euler Angles to Rotation Matrix (Relative YZX)/1
  Demux/3 -> Euler Angles to Rotation Matrix (Relative YZX)/2
  Demux/1 -> Euler Angles to Rotation Matrix (Relative YZX)/3

== system Mission_Server_QDrone_YOLO_Landing_Diagnostics/MISSION SERVER - LEADER//FOLLOWER with QBot 2e and QDrone/JOYSTICK/Pulse Check/pulse count  ==
  Trigger : TriggerPort  TriggerType=either  VariantControl=Variant
  Constant1 : Constant  Value=0
  Increment Stored Integer : simulink/Additional Math & Discrete/Additional Math: Increment - Decrement/Increment Stored Integer
  Sum : Sum  Inputs=|++
  Unit Delay : UnitDelay  SampleTime=-1  HasFrameUpgradeWarning=on
  Number of Pulses : Outport  VectorParamsAs1DForOutWhenUnconnected=off
  wires:
  Constant1/1 -> Sum/1
  Sum/1 -> Increment Stored Integer/1
  Unit Delay/1 -> Sum/2
  Increment Stored Integer/1 -> Unit Delay/1, Number of Pulses/1

== matlab function Mission_Server_QDrone_YOLO_Landing_Diagnostics/MISSION SERVER - LEADER//FOLLOWER with QBot 2e and QDrone/Grid Search Manager ==
  data: measuredPose input; desiredPose output; homePose input; triggers input; waypointIndex output; gridComplete output; visitedCount output; confirmedPad input; holdPose input; padU input; padV input; newPadSample input; centeringActive output; centered output; pixelError output; isTracking input; descentStage output; descentAbort output
function [desiredPose,waypointIndex,gridComplete,visitedCount,centeringActive,centered,pixelError,descentStage,descentAbort] = fcn(measuredPose,homePose,triggers,confirmedPad,holdPose,padU,padV,newPadSample,isTracking)
%#codegen
% Stage 0: search; 1: center at 0.70; 2: descend to 0.60;
% 3: center at 0.60; 4: descend to 0.55; 5: low hover.
persistent stage dwell takeoffWasLow reverseOrder complete visited sessionActive centerMode centerPose centerOrigin centerGood descentMode abortLatched
if isempty(stage)
 stage=uint8(0);dwell=uint16(0);takeoffWasLow=true;reverseOrder=false;
 complete=false;visited=uint8(0);sessionActive=false;centerMode=false;
 centerPose=zeros(4,1);centerOrigin=zeros(2,1);centerGood=uint8(0);
 descentMode=uint8(0);abortLatched=false;
end
takeoff=triggers(2)>0.5;
wps=[-1.2 -1 0.7;-0.6 -1 0.7;0 -1 0.7;0.6 -1 0.7;1.2 -1 0.7;1.2 -0.333333 0.7;0.6 -0.333333 0.7;0 -0.333333 0.7;-0.6 -0.333333 0.7;-1.2 -0.333333 0.7;-1.2 0.333333 0.7;-0.6 0.333333 0.7;0 0.333333 0.7;0.6 0.333333 0.7;1.2 0.333333 0.7;1.2 1 0.7;0.6 1 0.7;0 1 0.7;-0.6 1 0.7;-1.2 1 0.7];
baseMap=[0.00163 0.00019;7e-05 -0.00166];
cameraOffset=[0.11;0];
imageCenter=[320;240];
pixelError=zeros(2,1);
validPose=all(isfinite(measuredPose)) && all(isfinite(homePose));
if ~takeoff
 stage=uint8(0);dwell=uint16(0);takeoffWasLow=true;reverseOrder=false;
 sessionActive=false;centerMode=false;centerGood=uint8(0);
 descentMode=uint8(0);abortLatched=false;
elseif ~sessionActive
 complete=false;visited=uint8(0);sessionActive=true;
end
if takeoff && confirmedPad && isTracking>0.5 && validPose && ~centerMode
 centerMode=true;centerPose=holdPose;centerPose(3)=0.70;
 centerOrigin=holdPose(1:2);centerGood=uint8(0);descentMode=uint8(1);
end
desiredPose=homePose;desiredPose(3)=0.70;
if centerMode
 if isTracking<=0.5 || ~validPose || ~confirmedPad || measuredPose(3)<0.45
  abortLatched=true;centerGood=uint8(0);
  if validPose && isTracking>0.5
   centerPose(3)=min(max(measuredPose(3),0.55),0.70);
  end
 end
 if ~abortLatched
  h=min(max(measuredPose(3),0.50),0.70);
  map=baseMap*(h/0.70);
  target=imageCenter-map\cameraOffset;
  pixelError=[padU-target(1);padV-target(2)];
  if newPadSample
   if norm(pixelError)<=20
    if centerGood<uint8(10),centerGood=centerGood+uint8(1);end
   else
    centerGood=uint8(0);
    bodyStep=map*pixelError;
    a=measuredPose(4)-0.015;
    R=[cos(a) -sin(a);sin(a) cos(a)];
    step=R*bodyStep;n=norm(step);
    if n>0.005,step=step*(0.005/n);end
    candidate=centerPose(1:2)+step;
    offset=candidate-centerOrigin;on=norm(offset);
    if on>0.5,candidate=centerOrigin+offset*(0.5/on);end
    xLim=[-1.2 1.2];yLim=[-1 1];
    centerPose(1)=min(max(candidate(1),xLim(1)),xLim(2));
    centerPose(2)=min(max(candidate(2),yLim(1)),yLim(2));
   end
   xyError=norm(measuredPose(1:2)-centerPose(1:2));
   if centerGood>=uint8(10) && xyError<=0.12
    if descentMode==uint8(1) && abs(measuredPose(3)-0.70)<=0.05
     descentMode=uint8(2);centerPose(3)=0.60;centerGood=uint8(0);
    elseif descentMode==uint8(2) && abs(measuredPose(3)-0.60)<=0.05
     descentMode=uint8(3);centerGood=uint8(0);
    elseif descentMode==uint8(3) && abs(measuredPose(3)-0.60)<=0.05
     descentMode=uint8(4);centerPose(3)=0.55;centerGood=uint8(0);
    elseif descentMode==uint8(4) && abs(measuredPose(3)-0.55)<=0.05
     descentMode=uint8(5);centerGood=uint8(0);
    end
   end
  end
 end
 desiredPose=centerPose;
elseif takeoff && takeoffWasLow
 eHome=measuredPose(1:3)-desiredPose(1:3);
 if norm(eHome)<=0.12
  dwell=dwell+uint16(1);
  if dwell>=uint16(100)
   dFirst=measuredPose(1:2)-wps(1,1:2);
   dLast=measuredPose(1:2)-wps(20,1:2);
   reverseOrder=sum(dLast.*dLast)<sum(dFirst.*dFirst);
   stage=uint8(1);dwell=uint16(0);takeoffWasLow=false;
  end
 else,dwell=uint16(0);end
elseif takeoff && stage>=1
 idx=double(stage);if reverseOrder,idx=21-idx;end
 desiredPose(1:3)=wps(idx,:);
 e=measuredPose(1:3)-desiredPose(1:3);
 if norm(e)<=0.12
  dwell=dwell+uint16(1);
  if dwell>=uint16(100)
   visited=stage;
   if stage<uint8(20),stage=stage+uint8(1);else,complete=true;end
   dwell=uint16(0);
  end
 else,dwell=uint16(0);end
end
waypointIndex=0;
if stage>=uint8(1)
 waypointIndex=double(stage);if reverseOrder,waypointIndex=21-waypointIndex;end
end
gridComplete=complete;visitedCount=double(visited);
centeringActive=centerMode;centered=centerGood>=uint8(10) && descentMode==uint8(5);
descentStage=double(descentMode);descentAbort=abortLatched;
end

== matlab function Mission_Server_QDrone_YOLO_Landing_Diagnostics/MISSION SERVER - LEADER//FOLLOWER with QBot 2e and QDrone/Extract Vehicle Data - QDrone/Extract Object Data ==
  data: data input; position output; orientation output; index input; tracking output
function [position, orientation, tracking] = fcn(data, index)

n = length(data)/7;

if (index<=0)||(index>n)
    position = zeros(1,3); orientation = zeros(1,3); tracking = 0;
else
    position = [data(index*3-2), data(index*3-1), data(index*3)];
    orientation = [data((index+n)*3 - 2), data((index+n)*3 - 1), data((index+n)*3)];
    tracking = data(index + (n*6));
end

== matlab function Mission_Server_QDrone_YOLO_Landing_Diagnostics/Communication - QDrone/Detect Communication loss/MATLAB Function ==
  data: time input; stream_connection_loss output; state input; error input
function stream_connection_loss  = fcn(time, state, error)

stream_connection_loss = 0;
if time > 1
    if ~((state == 2)&&(error >= 0))
        % stream connection is not established correctly
        stream_connection_loss = 1;
    end
end

== matlab function Mission_Server_QDrone_YOLO_Landing_Diagnostics/MISSION SERVER - LEADER//FOLLOWER with QBot 2e and QDrone/YOLO Confirmation and Hover Hold ==
  data: measuredPose input; confirmedPad output; vision input; newVision input; clockTime input; triggers input; holdPose output; confidence output; padU output; padV output; newPadSample output; visionAge output
function [confirmedPad,holdPose,confidence,padU,padV,newPadSample,visionAge] = fcn(measuredPose,vision,newVision,clockTime,triggers)
%#codegen
persistent good bad active captured lastFrame lastFresh latestU latestV
if isempty(good), good=uint8(0); bad=uint8(0); active=false; captured=zeros(4,1); lastFrame=-1; lastFresh=-1; latestU=0; latestV=0; end
takeoff=triggers(2)>0.5; newPadSample=false;
if ~takeoff, good=uint8(0); bad=uint8(0); active=false; lastFresh=clockTime; end
if takeoff && newVision && vision(5)~=lastFrame
 lastFrame=vision(5); lastFresh=clockTime; valid=vision(1)>0.5 && vision(4)>=0.600000 && vision(2)>=0 && vision(2)<=640 && vision(3)>=0 && vision(3)<=480;
 if valid, latestU=vision(2); latestV=vision(3); newPadSample=true; bad=uint8(0); if good<uint8(5),good=good+uint8(1);end; if ~active && good>=uint8(5),active=true;captured=measuredPose;end
 else, good=uint8(0); if bad<uint8(10),bad=bad+uint8(1);end; if active && bad>=uint8(10),active=false;end; end
end
if active && (lastFresh<0 || clockTime-lastFresh>0.500000),active=false;good=uint8(0);bad=uint8(0);end
confirmedPad=active;holdPose=captured;confidence=vision(4);padU=latestU;padV=latestV;
if lastFresh<0,visionAge=Inf;else,visionAge=max(0,clockTime-lastFresh);end
end

== matlab function Mission_Server_QDrone_YOLO_Landing_Diagnostics/MISSION SERVER - LEADER//FOLLOWER with QBot 2e and QDrone/Landing Readiness Gate ==
  data: descentStage input; landingReady output; descentAbort input; confirmedPad input; centered input; newPadSample input; isTracking input; measuredPose input; desiredPose input; clockTime input; freshCount output; reasonCode output
function [landingReady,freshCount,reasonCode] = fcn(descentStage,descentAbort,confirmedPad,centered,newPadSample,isTracking,measuredPose,desiredPose,clockTime)
%#codegen
% Diagnostic only. This block never changes a Commander trigger or pose.
% Reason: 0 ready, 1 stage, 2 abort, 3 vision, 4 tracking/pose,
%         5 alignment/height, 6 stale, 7 accumulating fresh observations.
persistent count lastFresh
if isempty(count)
 count=uint8(0);lastFresh=-1;
end
landingReady=false;reasonCode=uint8(7);
if descentStage~=5
 count=uint8(0);lastFresh=-1;reasonCode=uint8(1);
elseif descentAbort>0.5
 count=uint8(0);lastFresh=-1;reasonCode=uint8(2);
elseif confirmedPad<=0.5
 count=uint8(0);lastFresh=-1;reasonCode=uint8(3);
elseif isTracking<=0.5 || ~all(isfinite(measuredPose)) || ~all(isfinite(desiredPose)) || ~isfinite(clockTime)
 count=uint8(0);lastFresh=-1;reasonCode=uint8(4);
elseif centered<=0.5 || norm(measuredPose(1:2)-desiredPose(1:2))>0.08 || abs(measuredPose(3)-0.55)>0.04
 count=uint8(0);lastFresh=-1;reasonCode=uint8(5);
elseif ~newPadSample && (lastFresh<0 || clockTime-lastFresh>0.50)
 count=uint8(0);lastFresh=-1;reasonCode=uint8(6);
else
 if newPadSample
  if lastFresh<0 || clockTime-lastFresh>0.50
   count=uint8(0);
  end
  lastFresh=clockTime;
  if count<uint8(10),count=count+uint8(1);end
 end
 landingReady=count>=uint8(10) && lastFresh>=0 && clockTime-lastFresh<=0.50;
 if landingReady,reasonCode=uint8(0);end
end
freshCount=double(count);
end

== matlab function Mission_Server_QDrone_YOLO_Landing_Diagnostics/MISSION SERVER - LEADER//FOLLOWER with QBot 2e and QDrone/Abort Diagnostic ==
  data: descentStage input; causeBits output; descentAbort input; confirmedPad input; isTracking input; measuredPose input; visionAge input; clockTime input; ageAtAbort output; timeAtAbort output
function [causeBits,ageAtAbort,timeAtAbort] = fcn(descentStage,descentAbort,confirmedPad,isTracking,measuredPose,visionAge,clockTime)
%#codegen
% Latch all conditions present at the first abort sample. Diagnostic only.
% Bits: 1 pad confirmation lost, 2 tracking lost, 4 invalid pose,
%       8 below 0.45 m, 16 abort with none of these inputs observed.
persistent seenAbort savedBits savedAge savedTime
if isempty(seenAbort)
 seenAbort=false;savedBits=0;savedAge=0;savedTime=0;
end
if descentStage==0 && descentAbort<=0.5
 seenAbort=false;savedBits=0;savedAge=0;savedTime=0;
elseif descentAbort>0.5 && ~seenAbort
 bits=0;
 if confirmedPad<=0.5,bits=bits+1;end
 if isTracking<=0.5,bits=bits+2;end
 if ~all(isfinite(measuredPose)),bits=bits+4;end
 if isfinite(measuredPose(3)) && measuredPose(3)<0.45,bits=bits+8;end
 if bits==0,bits=16;end
 savedBits=bits;savedAge=visionAge;savedTime=clockTime;seenAbort=true;
end
causeBits=savedBits;ageAtAbort=savedAge;timeAtAbort=savedTime;
end
